simulink model "six_stepItext"  (R2024a)
settings: Solver=ode23t  StartTime=0.0  StopTime=10  MaxStep=1e-6  RelTol=1e-4
undefined symbols (not defined in the file): DiscIntNeverNeededParam
libraries: simulink x24, nesl_utility x13, ee_lib x6, fl_lib x6, eePwmGenerator x1
(part 1 of 2)
settings Model: SimulationMode=accelerator  Creator=25415  LastModifiedBy=25415

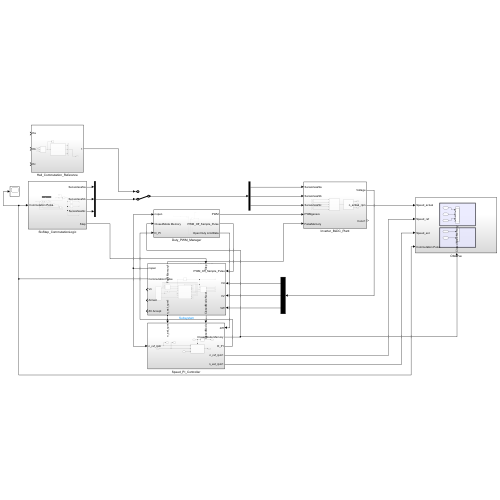
[thumbnail: Simulink's stored preview of the top-level diagram]
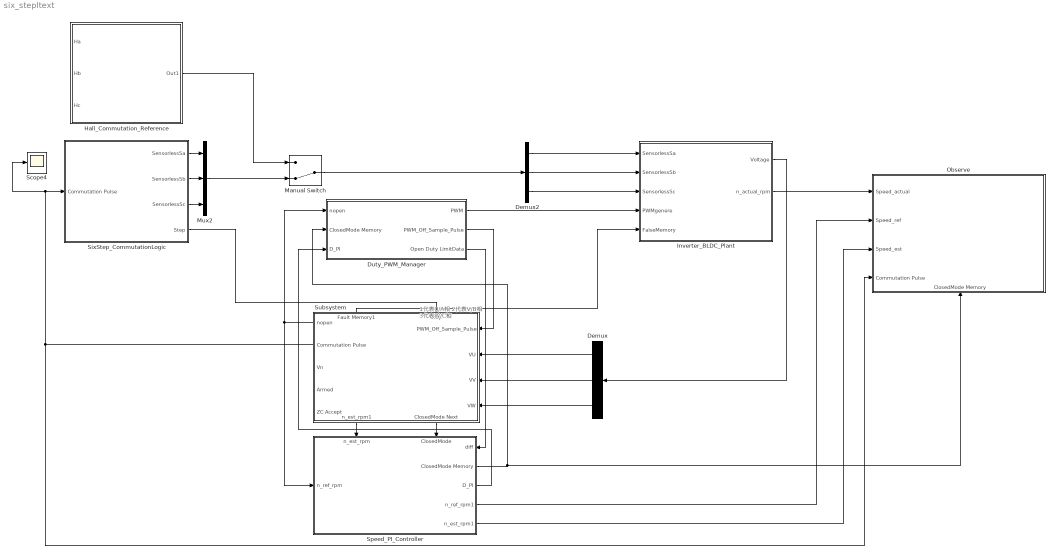
== system six_stepItext ==
  note: 1代表U/A相
      | 2代表V/B相
      | 3代表W/C相
  Demux : Demux  Outputs=3
  Demux2 : Demux  Outputs=3
  Duty_PWM_Manager : Subsystem
  Hall_Commutation_Reference : Subsystem
  Inverter_BLDC_Plant : Subsystem
  Manual Switch : ManualSwitch  CurrentSetting=0
  Mux2 : Mux  Inputs=3
  Observe : Subsystem
      settings: PortSchema="{\"entries\":[{\"content\":{\"sides\":[{\"content\":{\"connectorIds\":[\"In1\",\"In2\",\"In3\",\"In4\"]},\"type\":\"ConnectorPlacement.EquallySpacedRectSide\",\"uuid\":\"9088793b-2014-4196-a719-1ae128c634bd\"},{\"content\":{\"side\":\"RIGHT\"},\"type\":\"ConnectorPlacement.EquallySpacedRectSide\",\"uuid\":\"173c01ed-895e-413e-a79c-9815030dd1a7\"},{\"content\":{\"side\":\"TOP\"},\"type\":\"ConnectorPlacement.EquallySpacedRectSide\",\"uuid\":\"97f01aa3-a0bc-4305-9aad-804b5494463d\"},{\"content\":{\"connectorIds\":[\"In5\"],\"side\":\"BOTTOM\"},\"type\":\"ConnectorPlacement.EquallySpacedRectSide\",\"uuid\":\"39a9b1ee-11d5-4763-bc6a-eddc1daf8ee3\"}]},\"type\":\"ConnectorPlacement.EquallySpacedConnector\",\"uuid\":\"f0f9deaa-30fa-496c-8cff-10ccb2f5b2cf\"}],\"packageUris\":[\"http://schema.mathworks.com/mf0/Connector/R2020b\"],\"version\":\"1.0\"}"
  Scope4 : Scope
  SixStep_CommutationLogic : Subsystem
  Speed_PI_Controller : Subsystem
      settings: PortSchema="{\"entries\":[{\"content\":{\"sides\":[{\"content\":{\"connectorIds\":[\"In1\"]},\"type\":\"ConnectorPlacement.EquallySpacedRectSide\",\"uuid\":\"8a8ee2e6-da43-4c48-942d-e921ad8bcf3e\"},{\"content\":{\"connectorIds\":[\"In4\",\"Out1\",\"Out2\",\"Out3\",\"Out4\"],\"side\":\"RIGHT\"},\"type\":\"ConnectorPlacement.EquallySpacedRectSide\",\"uuid\":\"836c52b4-ac3a-4487-9ffc-d5efd4795786\"},{\"content\":{\"connectorIds\":[\"In2\",\"In3\"],\"side\":\"TOP\"},\"type\":\"ConnectorPlacement.EquallySpacedRectSide\",\"uuid\":\"5ec63cd2-cc9c-4304-9815-6f512e278e15\"},{\"content\":{\"side\":\"BOTTOM\"},\"type\":\"ConnectorPlacement.EquallySpacedRectSide\",\"uuid\":\"5132e6d1-af86-4b59-9d6a-b07b9b3af0b9\"}]},\"type\":\"ConnectorPlacement.EquallySpacedConnector\",\"uuid\":\"ac3d9a82-96c0-4f89-ae52-07d69004cd78\"}],\"packageUris\":[\"http://schema.mathworks.com/mf0/Connector/R2020b\"],\"version\":\"1.0\"}"
  Subsystem : Subsystem
      settings: PortSchema="{\"entries\":[{\"content\":{\"sides\":[{\"content\":{\"connectorIds\":[\"In1\",\"In2\",\"In3\",\"In4\"]},\"type\":\"ConnectorPlacement.EquallySpacedRectSide\",\"uuid\":\"0454e366-7b0d-4657-8f1b-5f34838f4f79\"},{\"content\":{\"connectorIds\":[\"Out1\",\"Out2\",\"Out3\",\"Out4\",\"Out5\"],\"side\":\"RIGHT\"},\"type\":\"ConnectorPlacement.EquallySpacedRectSide\",\"uuid\":\"85c00b62-bded-4496-b2c0-b773fc71ee5c\"},{\"content\":{\"connectorIds\":[\"In5\",\"Out8\"],\"side\":\"TOP\"},\"type\":\"ConnectorPlacement.EquallySpacedRectSide\",\"uuid\":\"3240dca5-fa46-4bda-9873-c5e2b8c1d629\"},{\"content\":{\"connectorIds\":[\"Out6\",\"Out7\"],\"side\":\"BOTTOM\"},\"type\":\"ConnectorPlacement.EquallySpacedRectSide\",\"uuid\":\"47798f7f-7eed-4b14-9289-d21656a674be\"}]},\"type\":\"ConnectorPlacement.EquallySpacedConnector\",\"uuid\":\"b9e37fa7-d7c3-43fc-b27e-fc50c7c41c36\"}],\"packageUris\":[\"http://schema.mathworks.com/mf0/Connector/R2020b\"],\"version\":\"1.0\"}"
  wires:
  SixStep_CommutationLogic/2(SensorlessSb) -> Mux2/2
  SixStep_CommutationLogic/1(SensorlessSa) -> Mux2/1
  SixStep_CommutationLogic/3(SensorlessSc) -> Mux2/3
  Mux2/1 -> Manual Switch/2
  Hall_Commutation_Reference/1(Out1) -> Manual Switch/1
  Manual Switch/1 -> Demux2/1
  Demux2/1 -> Inverter_BLDC_Plant/1(SensorlessSa)
  Demux2/2 -> Inverter_BLDC_Plant/2(SensorlessSb)
  Demux2/3 -> Inverter_BLDC_Plant/3(SensorlessSc)
  Inverter_BLDC_Plant/1(Voltage) -> Demux/1
  Duty_PWM_Manager/1(PWM) -> Inverter_BLDC_Plant/4(PWMgenere)
  Duty_PWM_Manager/3(Open Duty LimitData) -> Speed_PI_Controller/4(diff)
  Speed_PI_Controller/1(ClosedMode Memory) -> Observe/5(ClosedMode Memory), Duty_PWM_Manager/2(ClosedMode Memory)
  Speed_PI_Controller/2(D_PI) -> Duty_PWM_Manager/3(D_PI)
  Subsystem/2(Commutation Pulse) -> Scope4/1, SixStep_CommutationLogic/1(Commutation Pulse), Observe/4(Commutation Pulse)
  Subsystem/1(nopen) -> Duty_PWM_Manager/1(nopen), Speed_PI_Controller/1(n_ref_rpm)
  Duty_PWM_Manager/2(PWM_Off_Sample_Pulse) -> Subsystem/1(PWM_Off_Sample_Pulse)
  SixStep_CommutationLogic/4(Step) -> Subsystem/5(Step)
  Demux/1 -> Subsystem/2(VU)
  Demux/2 -> Subsystem/3(VV)
  Demux/3 -> Subsystem/4(VW)
  Subsystem/8(Fault Memory1) -> Inverter_BLDC_Plant/5(FalseMemory)
  Subsystem/6(ClosedMode Next) -> Speed_PI_Controller/3(ClosedMode)
  Subsystem/7(n_est_rpm1) -> Speed_PI_Controller/2(n_est_rpm)
  Speed_PI_Controller/3(n_ref_rpm1) -> Observe/2(Speed_ref)
  Speed_PI_Controller/4(n_est_rpm1) -> Observe/3(Speed_est)
  Inverter_BLDC_Plant/2(n_actual_rpm) -> Observe/1(Speed_actual)

== system six_stepItext/Duty_PWM_Manager ==
  nopen : Inport
  ClosedMode Memory : Inport  Port=2
  D_PI : Inport  Port=3
  Detect Decrease : simulink/Logic and Bit Operations/Detect Decrease  vinit=0.0  OutDataTypeStr=boolean
  Subsystem : Subsystem
  Subsystem3 : Subsystem
  Unit Delay : UnitDelay  SampleTime=10e-6  HasFrameUpgradeWarning=on
  Zero-Order Hold1 : ZeroOrderHold  SampleTime=10e-6
  PWM : Outport
  PWM_Off_Sample_Pulse : Outport  Port=2
  Open Duty LimitData : Outport  Port=3
  wires:
  D_PI/1 -> Subsystem3/3(D_PI)
  Subsystem3/1(PWM) -> PWM/1, Zero-Order Hold1/1
  ClosedMode Memory/1 -> Subsystem3/2(ClosedMode Memory)
  Subsystem/1(Open Duty LimitData) -> Open Duty LimitData/1, Subsystem3/1(In1)
  Zero-Order Hold1/1 -> Detect Decrease/1  "PWM_10us"
  Detect Decrease/1 -> Unit Delay/1
  nopen/1 -> Subsystem/1(nopen)
  Unit Delay/1 -> PWM_Off_Sample_Pulse/1  "PWM_Off_Sample_Pulse"

== system six_stepItext/Hall_Commutation_Reference ==
  Ha : Inport
  Hb : Inport  Port=2
  Hc : Inport  Port=3
  Hallencoder : Subsystem
  Mux1 : Mux  Inputs=3
  Scope2 : Scope
  Subsystem : Subsystem
  Out1 : Outport
  wires:
  Hb/1 -> Hallencoder/2(Hb)
  Subsystem/2(Sb) -> Mux1/2
  Subsystem/1(Sa) -> Mux1/1
  Mux1/1 -> Out1/1
  Hallencoder/1(Hallcode) -> Scope2/1, Subsystem/1(Hallcode)
  Hc/1 -> Hallencoder/3(Hc)
  Subsystem/3(Sc) -> Mux1/3
  Ha/1 -> Hallencoder/1(Ha)

== system six_stepItext/Inverter_BLDC_Plant ==
  SensorlessSa : Inport
  SensorlessSb : Inport  Port=2
  SensorlessSc : Inport  Port=3
  PWMgenere : Inport  Port=4
  FalseMemory : Inport  Port=5
  DriveSystem : Subsystem
  Subsystem2 : Subsystem
  Conn1 : PMIOPort  Side=Right
  Voltage : Outport
  n_actual_rpm : Outport  Port=2
  wires:
  SensorlessSc/1 -> DriveSystem/3(SensorlessSc)
  Subsystem2/1(Voltage) -> Voltage/1
  FalseMemory/1 -> DriveSystem/5(FalseMemory)
  PWMgenere/1 -> DriveSystem/4(PWMgenere)
  SensorlessSa/1 -> DriveSystem/1(SensorlessSa)
  SensorlessSb/1 -> DriveSystem/2(SensorlessSb)
  Subsystem2/2(n_actual_rpm) -> n_actual_rpm/1
  connections:
  Subsystem2/RConn1 -- Conn1/RConn1
  DriveSystem/RConn1 -- Subsystem2/LConn1

== system six_stepItext/Observe ==
  note: SpeedObserve
  note: StateObserve
  Speed_actual : Inport
  Speed_ref : Inport  Port=2
  Speed_est : Inport  Port=3
  Commutation Pulse : Inport  Port=4
  ClosedMode Memory : Inport  Port=5
  Scope : Scope  NumInputPorts=3
  Scope1 : Scope  NumInputPorts=2
  Scope2 : Scope  NumInputPorts=3
  wires:
  Speed_ref/1 -> Scope/1
  Speed_est/1 -> Scope/2
  Speed_actual/1 -> Scope/3
  Commutation Pulse/1 -> Scope1/1
  ClosedMode Memory/1 -> Scope1/2

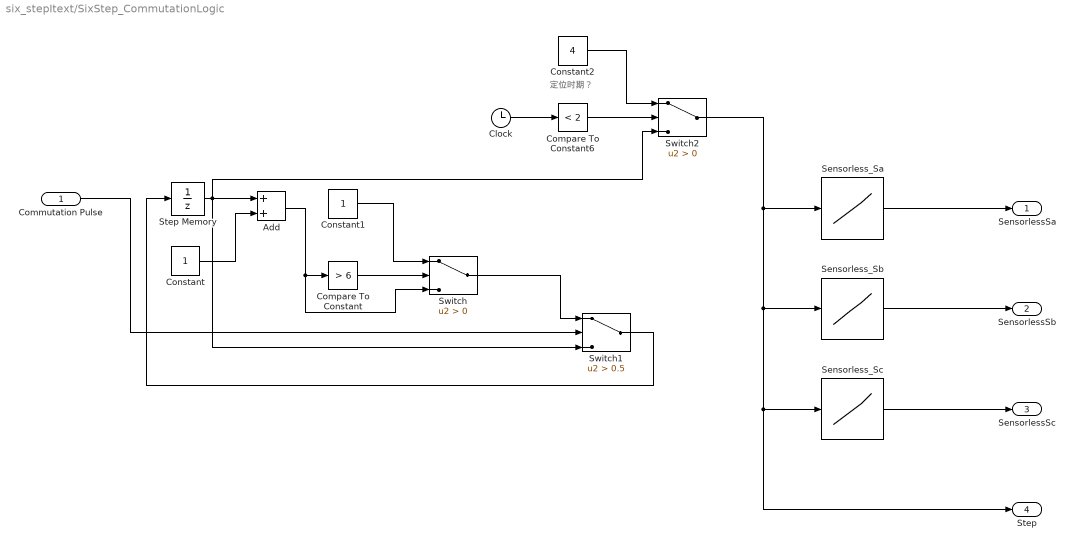
== system six_stepItext/SixStep_CommutationLogic ==
  note: 定位时期？
  Commutation Pulse : Inport
  Add : Sum
  Clock : Clock
  Compare To Constant : simulink/Logic and Bit Operations/Compare To Constant  relop=>  const=6  OutDataTypeStr=boolean
  Compare To Constant6 : simulink/Logic and Bit Operations/Compare To Constant  relop=<  const=2  OutDataTypeStr=boolean
  Constant : Constant
  Constant1 : Constant
  Constant2 : Constant  Value=4
  Sensorless_Sa : Lookup_n-D  NumberOfTableDimensions=1  BreakpointsForDimension1=[0 1 2 3 4 5 6]  Table=[0 -1 -1 0 1 1 0]  InterpMethod=Flat  InternalRulePriority=Speed  OutDataTypeStr=double  RndMeth=Simplest
  Sensorless_Sb : Lookup_n-D  NumberOfTableDimensions=1  BreakpointsForDimension1=[0 1 2 3 4 5 6]  Table=[0 1 0 -1 -1 0 1]  InterpMethod=Flat  InternalRulePriority=Speed  OutDataTypeStr=double  RndMeth=Simplest
  Sensorless_Sc : Lookup_n-D  NumberOfTableDimensions=1  BreakpointsForDimension1=[0 1 2 3 4 5 6]  Table=[0 0 1 1 0 -1 -1]  InterpMethod=Flat  InternalRulePriority=Speed  OutDataTypeStr=double  RndMeth=Simplest
  Step Memory : UnitDelay  InitialCondition=5  SampleTime=10e-6  HasFrameUpgradeWarning=on
  Switch : Switch  Criteria=u2 > Threshold  SaturateOnIntegerOverflow=off  InputSameDT=off
  Switch1 : Switch  Criteria=u2 > Threshold  Threshold=0.5  SaturateOnIntegerOverflow=off  InputSameDT=off
  Switch2 : Switch  Criteria=u2 > Threshold  SaturateOnIntegerOverflow=off  InputSameDT=off
  SensorlessSa : Outport
  SensorlessSb : Outport  Port=2
  SensorlessSc : Outport  Port=3
  Step : Outport  Port=4
  wires:
  Step Memory/1 -> Add/1, Switch2/3, Switch1/3
  Constant/1 -> Add/2
  Add/1 -> Switch/3, Compare To Constant/1
  Compare To Constant/1 -> Switch/2
  Constant1/1 -> Switch/1
  Commutation Pulse/1 -> Switch1/2
  Switch1/1 -> Step Memory/1
  Sensorless_Sa/1 -> SensorlessSa/1
  Sensorless_Sb/1 -> SensorlessSb/1
  Sensorless_Sc/1 -> SensorlessSc/1
  Clock/1 -> Compare To Constant6/1
  Compare To Constant6/1 -> Switch2/2
  Constant2/1 -> Switch2/1
  Switch/1 -> Switch1/1
  Switch2/1 -> Sensorless_Sa/1, Sensorless_Sb/1, Step/1, Sensorless_Sc/1

== system six_stepItext/Speed_PI_Controller ==
  n_ref_rpm : Inport
  n_est_rpm : Inport  Port=2
  ClosedMode : Inport  Port=3
  diff : Inport  Port=4
  ClosedMode Memory1 : UnitDelay  SampleTime=10e-6  HasFrameUpgradeWarning=on
  Enabled Subsystem : Subsystem  TreatAsAtomicUnit=on
  ClosedMode Memory : Outport
  D_PI : Outport  Port=2
  n_ref_rpm1 : Outport  Port=3
  n_est_rpm1 : Outport  Port=4
  wires:
  diff/1 -> Enabled Subsystem/3(diff)
  n_ref_rpm/1 -> n_ref_rpm1/1, Enabled Subsystem/1(n_ref_rpm)
  ClosedMode/1 -> ClosedMode Memory1/1, Enabled Subsystem/Enable
  Enabled Subsystem/1(D_PI) -> D_PI/1
  ClosedMode Memory1/1 -> ClosedMode Memory/1
  n_est_rpm/1 -> n_est_rpm1/1, Enabled Subsystem/2(n_fb_rpm)

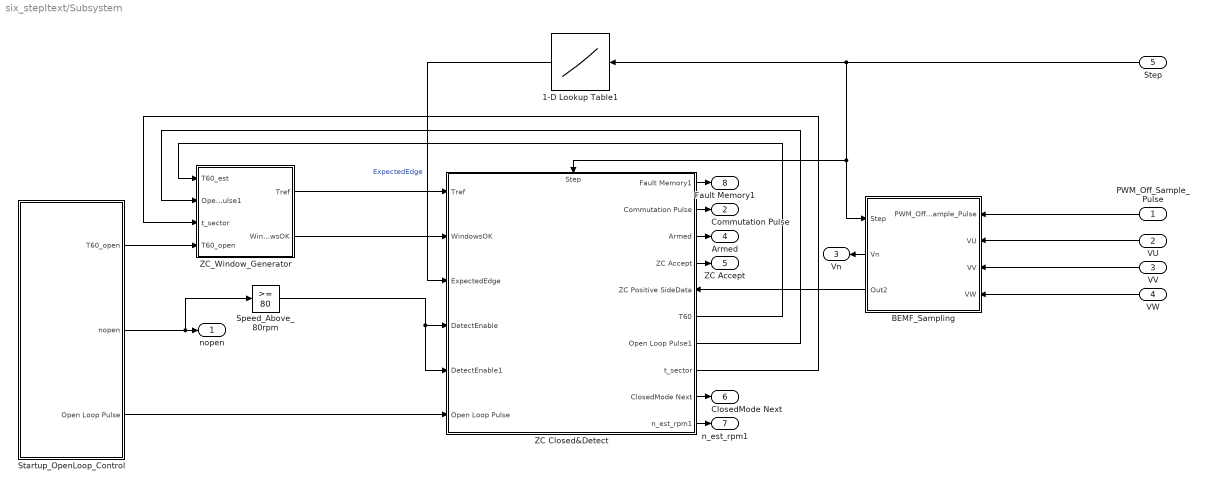
== system six_stepItext/Subsystem ==
  PWM_Off_Sample_Pulse : Inport
  VU : Inport  Port=2
  VV : Inport  Port=3
  VW : Inport  Port=4
  Step : Inport  Port=5
  1-D Lookup Table1 : Lookup_n-D  NumberOfTableDimensions=1  BreakpointsForDimension1=[0 1 2 3 4 5 6]  Table=[0 1 0 1 0 1 0]  InterpMethod=Flat  InternalRulePriority=Speed  RndMeth=Simplest
  BEMF_Sampling : Subsystem
      settings: PortSchema="{\"entries\":[{\"content\":{\"sides\":[{\"content\":{\"connectorIds\":[\"In1\",\"In2\",\"In3\",\"In4\"]},\"type\":\"ConnectorPlacement.EquallySpacedRectSide\",\"uuid\":\"219db874-4903-4521-ac7a-a4e5cace14e3\"},{\"content\":{\"connectorIds\":[\"In5\",\"Out1\",\"Out2\"],\"side\":\"RIGHT\"},\"type\":\"ConnectorPlacement.EquallySpacedRectSide\",\"uuid\":\"060f3999-5577-4659-ac56-31576aafd858\"},{\"content\":{\"side\":\"TOP\"},\"type\":\"ConnectorPlacement.EquallySpacedRectSide\",\"uuid\":\"b4eedb8b-4b2d-4953-a2bb-d0f589dd93bb\"}]},\"type\":\"ConnectorPlacement.EquallySpacedConnector\",\"uuid\":\"c9675ca2-e6a6-43e7-bc9f-5a6e20bc96da\"}],\"packageUris\":[\"http://schema.mathworks.com/mf0/Connector/R2020b\"],\"version\":\"1.0\"}"
  Speed_Above_80rpm : simulink/Logic and Bit Operations/Compare To Constant  relop=>=  const=80  OutDataTypeStr=boolean
  Startup_OpenLoop_Control : Subsystem
  ZC Closed&Detect : Subsystem
      settings: PortSchema="{\"entries\":[{\"content\":{\"sides\":[{\"content\":{\"connectorIds\":[\"In1\",\"In2\",\"In3\",\"In4\",\"In5\",\"In6\"]},\"type\":\"ConnectorPlacement.EquallySpacedRectSide\",\"uuid\":\"236afadc-2b12-4f95-9b78-5ff144fef5c1\"},{\"content\":{\"connectorIds\":[\"Out1\",\"Out2\",\"Out3\",\"Out4\",\"In8\",\"Out5\",\"Out6\",\"Out7\",\"Out8\",\"Out9\"],\"side\":\"RIGHT\"},\"type\":\"ConnectorPlacement.EquallySpacedRectSide\",\"uuid\":\"406734ed-d81f-414f-95f5-b90d5cc47299\"},{\"content\":{\"connectorIds\":[\"In7\"],\"side\":\"TOP\"},\"type\":\"ConnectorPlacement.EquallySpacedRectSide\",\"uuid\":\"56c21215-f7ac-4aca-9a8a-3ea4f76aa518\"}]},\"type\":\"ConnectorPlacement.EquallySpacedConnector\",\"uuid\":\"992103e6-5b89-45d8-b138-c7ecb7c3dad5\"}],\"packageUris\":[\"http://schema.mathworks.com/mf0/Connector/R2020b\"],\"version\":\"1.0\"}"
  ZC_Window_Generator : Subsystem
  nopen : Outport
  Commutation Pulse : Outport  Port=2
  Vn : Outport  Port=3
  Armed : Outport  Port=4
  ZC Accept : Outport  Port=5
  ClosedMode Next : Outport  Port=6
  n_est_rpm1 : Outport  Port=7
  Fault Memory1 : Outport  Port=8
  wires:
  ZC_Window_Generator/2(WindowsOK) -> ZC Closed&Detect/2(WindowsOK)
  Step/1 -> BEMF_Sampling/5(Step), ZC Closed&Detect/7(Step), 1-D Lookup Table1/1
  BEMF_Sampling/1(Vn) -> Vn/1
  ZC Closed&Detect/5(T60) -> ZC_Window_Generator/1(T60_est)
  Startup_OpenLoop_Control/1(T60_open) -> ZC_Window_Generator/4(T60_open)
  BEMF_Sampling/2(Out2) -> ZC Closed&Detect/8(ZC Positive SideData)
  Startup_OpenLoop_Control/3(Open Loop Pulse) -> ZC Closed&Detect/6(Open Loop Pulse)
  ZC Closed&Detect/7(t_sector) -> ZC_Window_Generator/3(t_sector)
  1-D Lookup Table1/1 -> ZC Closed&Detect/3(ExpectedEdge)  "ExpectedEdge"
  ZC Closed&Detect/9(n_est_rpm1) -> n_est_rpm1/1
  ZC Closed&Detect/6(Open Loop Pulse1) -> ZC_Window_Generator/2(Open Loop Pulse1)
  ZC_Window_Generator/1(Tref) -> ZC Closed&Detect/1(Tref)
  VW/1 -> BEMF_Sampling/4(VW)
  VU/1 -> BEMF_Sampling/2(VU)
  PWM_Off_Sample_Pulse/1 -> BEMF_Sampling/1(PWM_Off_Sample_Pulse)
  VV/1 -> BEMF_Sampling/3(VV)
  ZC Closed&Detect/2(Commutation Pulse) -> Commutation Pulse/1
  Startup_OpenLoop_Control/2(nopen) -> Speed_Above_80rpm/1, nopen/1
  ZC Closed&Detect/8(ClosedMode Next) -> ClosedMode Next/1
  ZC Closed&Detect/1(Fault Memory1) -> Fault Memory1/1
  ZC Closed&Detect/3(Armed) -> Armed/1
  ZC Closed&Detect/4(ZC Accept) -> ZC Accept/1
  Speed_Above_80rpm/1 -> ZC Closed&Detect/5(DetectEnable1), ZC Closed&Detect/4(DetectEnable)

== system six_stepItext/Duty_PWM_Manager/Subsystem ==
  nopen : Inport
  Add : Sum
  Divide : Product  Inputs=*/
  Open DC Voltage : Constant  Value=12
  Open Duty Limit : Saturate  UpperLimit=0.45  LowerLimit=0
  Open EMF Voltage : Gain  Gain=0.032
  Open Voltage Boost : Constant  Value=0.4
  Open Duty LimitData : Outport
  wires:
  Divide/1 -> Open Duty Limit/1
  Open DC Voltage/1 -> Divide/2
  Add/1 -> Divide/1
  Open Voltage Boost/1 -> Add/2
  Open EMF Voltage/1 -> Add/1
  Open Duty Limit/1 -> Open Duty LimitData/1
  nopen/1 -> Open EMF Voltage/1

== system six_stepItext/Duty_PWM_Manager/Subsystem3 ==
  In1 : Inport
  ClosedMode Memory : Inport  Port=2
  D_PI : Inport  Port=3
  Clock : Clock
  Compare To Constant7 : simulink/Logic and Bit Operations/Compare To Constant  relop=<  const=2  OutDataTypeStr=boolean
  Constant : Constant  Value=0.05
  PWM Generator : eePwmGenerator/PWM Generator  CarrCount=Up  Tper=50e-6  Tdelay=0  Ts=1e-6
  Subsystem2 : Subsystem
  Switch1 : Switch  Criteria=u2 > Threshold  SaturateOnIntegerOverflow=off  InputSameDT=off
  PWM : Outport
  wires:
  Constant/1 -> Switch1/1
  D_PI/1 -> Subsystem2/1(D_PI)
  Switch1/1 -> Subsystem2/3(Duty)
  Clock/1 -> Compare To Constant7/1
  Compare To Constant7/1 -> Switch1/2
  ClosedMode Memory/1 -> Subsystem2/2(ClosedMode Memory)
  Subsystem2/1(PWM Generator) -> PWM Generator/1
  In1/1 -> Switch1/3
  PWM Generator/1 -> PWM/1

== system six_stepItext/Hall_Commutation_Reference/Hallencoder ==
  Ha : Inport
  Hb : Inport  Port=2
  Hc : Inport  Port=3
  Add : Sum  Inputs=+++
  Gain : Gain  Gain=4
  Gain1 : Gain  Gain=2
  Gain2 : Gain
  Hallcode : Outport
  wires:
  Ha/1 -> Gain/1
  Hc/1 -> Gain2/1
  Hb/1 -> Gain1/1
  Gain/1 -> Add/1
  Gain1/1 -> Add/2
  Gain2/1 -> Add/3
  Add/1 -> Hallcode/1

== system six_stepItext/Hall_Commutation_Reference/Subsystem ==
  Hallcode : Inport
  1-D Lookup Table : Lookup_n-D  NumberOfTableDimensions=1  BreakpointsForDimension1=[0 1 2 3 4 5 6 7]  Table=[0 0 -1 -1 1 1 0 0]  InterpMethod=Flat  InternalRulePriority=Speed  OutDataTypeStr=double  RndMeth=Simplest
  1-D Lookup Table1 : Lookup_n-D  NumberOfTableDimensions=1  BreakpointsForDimension1=[0 1 2 3 4 5 6 7]  Table=[0 -1 1 0 0 -1 1 0]  InterpMethod=Flat  InternalRulePriority=Speed  OutDataTypeStr=double  RndMeth=Simplest
  1-D Lookup Table2 : Lookup_n-D  NumberOfTableDimensions=1  BreakpointsForDimension1=[0 1 2 3 4 5 6 7]  Table=[0 1 0 1 -1 0 -1 0]  InterpMethod=Flat  InternalRulePriority=Speed  OutDataTypeStr=double  RndMeth=Simplest
  Sa : Outport
  Sb : Outport  Port=2
  Sc : Outport  Port=3
  wires:
  Hallcode/1 -> 1-D Lookup Table2/1, 1-D Lookup Table1/1, 1-D Lookup Table/1
  1-D Lookup Table/1 -> Sa/1
  1-D Lookup Table1/1 -> Sb/1
  1-D Lookup Table2/1 -> Sc/1

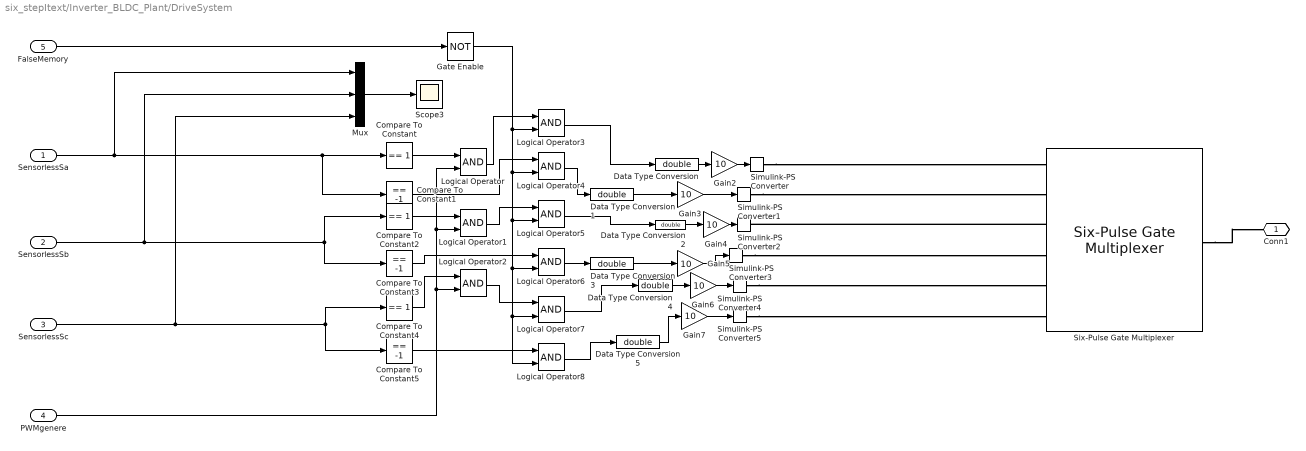
== system six_stepItext/Inverter_BLDC_Plant/DriveSystem ==
  SensorlessSa : Inport
  SensorlessSb : Inport  Port=2
  SensorlessSc : Inport  Port=3
  PWMgenere : Inport  Port=4
  FalseMemory : Inport  Port=5
  Compare To Constant : simulink/Logic and Bit Operations/Compare To Constant  relop===  const=1  OutDataTypeStr=boolean
  Compare To Constant1 : simulink/Logic and Bit Operations/Compare To Constant  relop===  const=-1  OutDataTypeStr=boolean
  Compare To Constant2 : simulink/Logic and Bit Operations/Compare To Constant  relop===  const=1  OutDataTypeStr=boolean
  Compare To Constant3 : simulink/Logic and Bit Operations/Compare To Constant  relop===  const=-1  OutDataTypeStr=boolean
  Compare To Constant4 : simulink/Logic and Bit Operations/Compare To Constant  relop===  const=1  OutDataTypeStr=boolean
  Compare To Constant5 : simulink/Logic and Bit Operations/Compare To Constant  relop===  const=-1  OutDataTypeStr=boolean
  Data Type Conversion{,1..5} (6 alike) : DataTypeConversion  OutDataTypeStr=double  SaturateOnIntegerOverflow=off  RndMeth=Floor
  Gain{2..7} (6 alike) : Gain  Gain=10
  Gate Enable : Logic  Operator=NOT  AllPortsSameDT=off  OutDataTypeStr=boolean
  Logical Operator{,1..8} (9 alike) : Logic  AllPortsSameDT=off  OutDataTypeStr=boolean
  Mux : Mux  Inputs=3
  Scope3 : Scope
  Simulink-PS Converter{,1..5} (6 alike) : nesl_utility/Simulink-PS Converter  PhysicalDomain=network_engine_domain  SubClassName=ps_input  LeftPortType=input  RightPortType=output  PseudoPeriodic=off  Frequencies=[]  NoiseDistribution=none  NoiseParameters=[]  Unit=V  AffineConversion=off  FilteringAndDerivatives=zero  SimscapeFilterOrder=1  InputFilterTimeConstant=0.001  UdotUserProvided=0
  Six-Pulse Gate Multiplexer : ee_lib/Semiconductors & Converters/Converters/Six-Pulse Gate Multiplexer  port_option=ee.enum.controlport.ps
  Conn1 : PMIOPort  Side=Right
  wires:
  Gain3/1 -> Simulink-PS Converter1/1
  SensorlessSb/1 -> Mux/2, Compare To Constant3/1, Compare To Constant2/1
  Data Type Conversion4/1 -> Gain6/1
  PWMgenere/1 -> Logical Operator1/2, Logical Operator/2, Logical Operator2/2
  SensorlessSc/1 -> Mux/3, Compare To Constant5/1, Compare To Constant4/1
  Gain2/1 -> Simulink-PS Converter/1
  Data Type Conversion5/1 -> Gain7/1
  Gain4/1 -> Simulink-PS Converter2/1
  Compare To Constant4/1 -> Logical Operator2/1
  Gain5/1 -> Simulink-PS Converter3/1
  Data Type Conversion3/1 -> Gain5/1
  Gain6/1 -> Simulink-PS Converter4/1
  Compare To Constant2/1 -> Logical Operator1/1
  Data Type Conversion/1 -> Gain2/1
  Mux/1 -> Scope3/1
  Data Type Conversion1/1 -> Gain3/1
  Data Type Conversion2/1 -> Gain4/1
  FalseMemory/1 -> Gate Enable/1
  SensorlessSa/1 -> Mux/1, Compare To Constant1/1, Compare To Constant/1
  Compare To Constant/1 -> Logical Operator/1
  Gain7/1 -> Simulink-PS Converter5/1
  Gate Enable/1 -> Logical Operator3/2, Logical Operator4/2, Logical Operator5/2, Logical Operator6/2, Logical Operator7/2, Logical Operator8/2
  Compare To Constant5/1 -> Logical Operator8/1
  Logical Operator8/1 -> Data Type Conversion5/1
  Logical Operator2/1 -> Logical Operator7/1
  Logical Operator7/1 -> Data Type Conversion4/1
  Logical Operator6/1 -> Data Type Conversion3/1
  Compare To Constant3/1 -> Logical Operator6/1
  Logical Operator1/1 -> Logical Operator5/1
  Compare To Constant1/1 -> Logical Operator4/1
  Logical Operator/1 -> Logical Operator3/1
  Logical Operator3/1 -> Data Type Conversion/1
  Logical Operator4/1 -> Data Type Conversion1/1
  Logical Operator5/1 -> Data Type Conversion2/1
  connections:
  Simulink-PS Converter1/RConn1 -- Six-Pulse Gate Multiplexer/LConn2
  Six-Pulse Gate Multiplexer/LConn3 -- Simulink-PS Converter2/RConn1
  Simulink-PS Converter/RConn1 -- Six-Pulse Gate Multiplexer/LConn1
  Simulink-PS Converter3/RConn1 -- Six-Pulse Gate Multiplexer/LConn4
  Simulink-PS Converter4/RConn1 -- Six-Pulse Gate Multiplexer/LConn5
  Simulink-PS Converter5/RConn1 -- Six-Pulse Gate Multiplexer/LConn6
  Six-Pulse Gate Multiplexer/RConn1 -- Conn1/RConn1

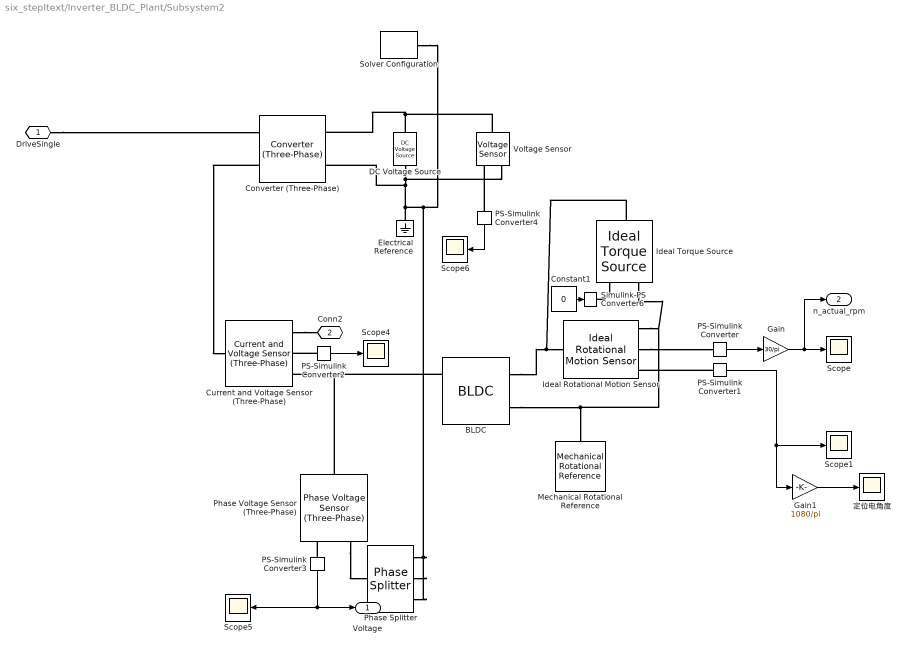
== system six_stepItext/Inverter_BLDC_Plant/Subsystem2 ==
  BLDC : ee_lib/Electromechanical/Permanent Magnet/BLDC  port_option=ee.enum.threePhasePort.composite  rotor_param=ee.enum.pmsm.backemf.trapezoidflux  pm_flux_linkage=0.03 Wb  theta_constant=pi / 12 rad  emf_max=9.6 V  w_meas=600 rpm  DphiDtheta_tab=[0, -.1528, -.1528, .1528, .1528, 0] Wb/rad  back_emf_tab=[0, -9.6, -9.6, 9.6, 9.6, 0] V  rotor_angle_tab=[0, 7.5, 22.5, 37.5, 52.5, 60] deg  nPolePairs=6  axes_param=ee.enum.rotorangle.daxis  winding_type=ee.enum.electromech.statorconfiguration.wye  stator_param=ee.enum.statorparam.LdLqL0  machine_param=ee.enum.dqparameterization.constant  Ld=0.00022 H  Lq=0.00022 H  idVec=[-200, 0, 200] A  iqVec=[-200, 0, 200] A  LdMatrix=0.00022 * ones(3, 3) H  LqMatrix=0.00022 * ones(3, 3) H  L0=0.00016 H  Ls=0.0002 H  Lm=0 H  Ms=0.00002 H  Rs=0.013 Ohm  zero_sequence=ee.enum.park.zerosequence.include  loss_param=ee.enum.ironloss.none  losses_oc=[0, 0, 0] W  losses_sc=[0, 0, 0] W  f_losses=60 Hz  Isc_losses=95 A  J=0.01 kg*m^2  lam=0.05 N*m*s/rad  i_d_specify=off  i_d_priority=None  i_d=0 A  i_d_nominal_specify=off  i_d_nominal_value=1  i_d_nominal_unit=A  i_q_specify=off  i_q_priority=None  i_q=0 A  i_q_nominal_specify=off  i_q_nominal_value=1  i_q_nominal_unit=A  torque_specify=off  torque_priority=None  torque=0 N*m  torque_nominal_specify=off  torque_nominal_value=1  torque_nominal_unit=N*m  angular_velocity_specify=off  angular_velocity_priority=High  angular_velocity=0 rpm  angular_velocity_nominal_specify=off  angular_velocity_nominal_value=1  angular_velocity_nominal_unit=rpm  angular_position_specify=off  angular_position_priority=High  angular_position=0 deg  angular_position_nominal_specify=off  angular_position_nominal_value=1  angular_position_nominal_unit=deg  alpha=3.93e-3 1/K  alpha_flux=-0.001 1/K  Tmeas=298.15 K  stator_thermal_mass=100 J/K  rotor_thermal_mass=200 J/K  Rm_percent_rotor=90  Rd_percent_rotor=30  temperatureA_specify=off  temperatureA_priority=High  temperatureA=25 degC  temperatureA_nominal_specify=off  temperatureA_nominal_value=1  temperatureA_nominal_unit=degC  temperatureB_specify=off  temperatureB_priority=High  temperatureB=25 degC  temperatureB_nominal_specify=off  temperatureB_nominal_value=1  temperatureB_nominal_unit=degC  temperatureC_specify=off  temperatureC_priority=High  temperatureC=25 degC  temperatureC_nominal_specify=off  temperatureC_nominal_value=1  temperatureC_nominal_unit=degC  temperatureR_specify=off  temperatureR_priority=High  temperatureR=25 degC  temperatureR_nominal_specify=off  temperatureR_nominal_value=1  temperatureR_nominal_unit=degC
      settings: InternalSimscapePortConfiguration="{\"Bottom\":[],\"Left\":[{\"id\":\"N\",\"label\":\"~\",\"type\":\"foundation.electrical.three_phase\"},{\"id\":\"n\",\"label\":\"n\",\"type\":\"foundation.electrical.electrical\"}],\"Right\":[{\"id\":\"R\",\"label\":\"R\",\"type\":\"foundation.mechanical.rotational.rotational\"},{\"id\":\"C\",\"label\":\"C\",\"type\":\"foundation.mechanical.rotational.rotational\"}],\"Top\":[]}"
  Constant1 : Constant  Value=0
  Converter (Three-Phase) : ee_lib/Semiconductors & Converters/Converters/Converter (Three-Phase)  port_option=ee.enum.threePhasePort.composite  fidelity_option=ee.enum.converters.fidelity.detailed  device_type=ee.enum.converters.switchingdevice.ideal  K=0  Vf=0.8 V  Ron=0.001 Ohm  Rds=0.001 Ohm  Goff=1e-6 1/Ohm  Vgt=1 V  Vgt_off=-1 V  Ih=1 A  Vth=6 V  diode_param=ee.enum.converters.protectiondiode.nodynamics  diode_Vf=0.8 V  diode_Ron=0.001 Ohm  diode_Goff=1e-5 1/Ohm  diode_C=50 nF  diode_iRM=-235 A  diode_iF=300 A  diode_idot=-50 A/us  diode_trr_param=ee.enum.converters.diodetrr.trr_factor  diode_trr_factor=3  diode_trr=15 us  diode_Qrr=1500 s*uA  snubber_type=ee.enum.converters.snubber.exclude  Cs=1e-7 F  Rs=0.1 Ohm
  Current and Voltage Sensor (Three-Phase) : ee_lib/Sensors & Transducers/Current and Voltage Sensor (Three-Phase)  vMeasurementType=ee.enum.vmeasurement.ll  outputUnit=ee.enum.unit.si  SRated=100e6 A*V  VRated=24e3 V  I_specify=off  I_priority=None  I=[0, 0, 0] A  I_nominal_specify=off  I_nominal_value=1  I_nominal_unit=A  V_specify=off  V_priority=None  V=[0, 0, 0] V  V_nominal_specify=off  V_nominal_value=1  V_nominal_unit=V
      settings: InternalSimscapePortConfiguration="{\"Bottom\":[],\"Left\":[{\"id\":\"N1\",\"label\":\"~1\",\"type\":\"foundation.electrical.three_phase\"}],\"Right\":[{\"id\":\"V_output\",\"label\":\"V\",\"type\":\"output\"},{\"id\":\"I_output\",\"label\":\"I\",\"type\":\"output\"},{\"id\":\"N2\",\"label\":\"~2\",\"type\":\"foundation.electrical.three_phase\"}],\"Top\":[]}"
  DC Voltage Source : fl_lib/Electrical/Electrical Sources/DC Voltage Source  v0=12 V
  Electrical Reference : fl_lib/Electrical/Electrical Elements/Electrical Reference
  Gain : Gain  Gain=30/pi
  Gain1 : Gain  Gain=1080/pi
  Ideal Rotational Motion Sensor : fl_lib/Mechanical/Mechanical Sensors/Ideal Rotational Motion Sensor  reference=foundation.enum.MeasurementReference.difference  acceleration_port=false  velocity_port=true  position_port=true  wrap_angle=false  offset=0 rad
  Ideal Torque Source : fl_lib/Mechanical/Mechanical Sources/Ideal Torque Source
  Mechanical Rotational Reference : fl_lib/Mechanical/Rotational Elements/Mechanical Rotational Reference
  PS-Simulink Converter : nesl_utility/PS-Simulink Converter  PhysicalDomain=network_engine_domain  SubClassName=ps_output  LeftPortType=input  RightPortType=output  PseudoPeriodic=off  Frequencies=[]  VectorFormat=inherit  Unit=rad/s  AffineConversion=off
  PS-Simulink Converter1 : nesl_utility/PS-Simulink Converter  PhysicalDomain=network_engine_domain  SubClassName=ps_output  LeftPortType=input  RightPortType=output  PseudoPeriodic=off  Frequencies=[]  VectorFormat=inherit  Unit=rad  AffineConversion=off
  PS-Simulink Converter2 : nesl_utility/PS-Simulink Converter  PhysicalDomain=network_engine_domain  SubClassName=ps_output  LeftPortType=input  RightPortType=output  PseudoPeriodic=off  Frequencies=[]  VectorFormat=inherit  Unit=A  AffineConversion=off
  PS-Simulink Converter3 : nesl_utility/PS-Simulink Converter  PhysicalDomain=network_engine_domain  SubClassName=ps_output  LeftPortType=input  RightPortType=output  PseudoPeriodic=off  Frequencies=[]  VectorFormat=inherit  Unit=V  AffineConversion=off
  PS-Simulink Converter4 : nesl_utility/PS-Simulink Converter  PhysicalDomain=network_engine_domain  SubClassName=ps_output  LeftPortType=input  RightPortType=output  PseudoPeriodic=off  Frequencies=[]  VectorFormat=inherit  Unit=V  AffineConversion=off
  Phase Splitter : ee_lib/Connectors & References/Phase Splitter
  Phase Voltage Sensor (Three-Phase) : ee_lib/Sensors & Transducers/Phase Voltage Sensor (Three-Phase)
  Scope{,1,4..6} (5 alike) : Scope
  Simulink-PS Converter6 : nesl_utility/Simulink-PS Converter  PhysicalDomain=network_engine_domain  SubClassName=ps_input  LeftPortType=input  RightPortType=output  PseudoPeriodic=off  Frequencies=[]  NoiseDistribution=none  NoiseParameters=[]  Unit=N*m  AffineConversion=off  FilteringAndDerivatives=zero  SimscapeFilterOrder=1  InputFilterTimeConstant=0.001  UdotUserProvided=0
  Solver Configuration : nesl_utility/Solver Configuration  PhysicalDomain=network_engine_domain  SubClassName=solver  LeftPortType=input  RightPortType=generic  Tones=[]  Harmonics=[]  SimulateNoise=off  Profile=off  UseLocalSampling=off  EnableSwitchedLinearOptims=on  FrequencyDomain=off  UseCCode=off  RelTol=0.001  AbsTol=0.001  MinStep=1e-09  ToWorkspace=off  RevertToSquareIcSolve=off  NumHomotopyIterations=100  PhasorMode=off  PhasorModeNumHarmonics=1  ConsistencySolver=NEWTON_XTOL_AFTER_FTOL  IndexReductionMethod=DerivativeReplacement  DoDC=off  ResidualTolerance=1e-09  ConsistencyTolSource=GLOBAL  ConsistencyAbsTol=0.001  ConsistencyRelTol=0.001  ConsistencyTolFactor=0.001  UseLocalSolver=off  LocalSolverChoice=NE_BACKWARD_EULER_ADVANCER  ResolveIndetEquations=on  FunctionEvalNumThread=1  LocalSolverSampleTime=0.001  DoFixedCost=off  MaxNonlinIter=3  MaxModeIter=2  ComputeImpulses=off  ImpulseIterations=2  LinearAlgebra=auto  LinearAlgebraNumThread=0  EquationFormulation=NE_TIME_EF  DelaysMemoryBudget=1024  AutomaticFiltering=on  FilteringTimeConstant=0.001  PartitionStorageMethod=AS_NEEDED  PartitionMemoryBudget=1024  PartitionMethod=ROBUST  MultibodyUseLocalSolver=off  MultibodyLocalSolverChoice=ODE1  MultibodyLocalSolverSampleTime=0.001
  Voltage Sensor : fl_lib/Electrical/Electrical Sensors/Voltage Sensor
  定位电角度 : Scope
  DriveSingle : PMIOPort  Side=Left
  Conn2 : PMIOPort  Port=2  Side=Right
  Voltage : Outport
  n_actual_rpm : Outport  Port=2
  wires:
  PS-Simulink Converter4/1 -> Scope6/1
  PS-Simulink Converter/1 -> Gain/1
  Constant1/1 -> Simulink-PS Converter6/1
  Gain/1 -> n_actual_rpm/1, Scope/1
  PS-Simulink Converter1/1 -> Gain1/1, Scope1/1
  PS-Simulink Converter2/1 -> Scope4/1
  PS-Simulink Converter3/1 -> Voltage/1, Scope5/1
  Gain1/1 -> 定位电角度/1
  connections:
  PS-Simulink Converter3/LConn1 -- Phase Voltage Sensor (Three-Phase)/RConn1
  DC Voltage Source/RConn1 -- Voltage Sensor/RConn2 -- Solver Configuration/RConn1 -- Phase Splitter/RConn3 -- Phase Splitter/RConn2 -- Phase Splitter/RConn1 -- Electrical Reference/LConn1 -- Converter (Three-Phase)/RConn2
  Current and Voltage Sensor (Three-Phase)/RConn1 -- Conn2/RConn1
  BLDC/RConn2 -- Ideal Torque Source/RConn2 -- Ideal Rotational Motion Sensor/RConn1 -- Mechanical Rotational Reference/LConn1
  PS-Simulink Converter1/LConn1 -- Ideal Rotational Motion Sensor/RConn3
  Converter (Three-Phase)/LConn2 -- Current and Voltage Sensor (Three-Phase)/LConn1
  BLDC/LConn1 -- Phase Voltage Sensor (Three-Phase)/LConn1 -- Current and Voltage Sensor (Three-Phase)/RConn3
  DC Voltage Source/LConn1 -- Voltage Sensor/LConn1 -- Converter (Three-Phase)/RConn1
  Phase Voltage Sensor (Three-Phase)/RConn2 -- Phase Splitter/LConn1
  BLDC/RConn1 -- Ideal Torque Source/LConn1 -- Ideal Rotational Motion Sensor/LConn1
  Ideal Rotational Motion Sensor/RConn2 -- PS-Simulink Converter/LConn1
  Ideal Torque Source/RConn1 -- Simulink-PS Converter6/RConn1
  PS-Simulink Converter4/LConn1 -- Voltage Sensor/RConn1
  PS-Simulink Converter2/LConn1 -- Current and Voltage Sensor (Three-Phase)/RConn2
  DriveSingle/RConn1 -- Converter (Three-Phase)/LConn1

== system six_stepItext/Speed_PI_Controller/Enabled Subsystem ==
  n_ref_rpm : Inport
  n_fb_rpm : Inport  Port=2
  diff : Inport  Port=3
  Enable : EnablePort  StatesWhenEnabling=reset
  Add : Sum  Inputs=+-
  Add1 : Sum  Inputs=+++
  Add2 : Sum
  Discrete-Time Integrator1 : DiscreteIntegrator  SampleTime=1e-3  LimitOutput=on  UpperSaturationLimit=0.3  LowerSaturationLimit=-0.3  ICPrevOutput=DiscIntNeverNeededParam  ICPrevScaledInput=DiscIntNeverNeededParam
  KI : Gain  Gain=0.005
  KP : Gain  Gain=0.001
  Kaw : Gain  Gain=5
  Saturation : Saturate  UpperLimit=0.45  LowerLimit=0
  Saturation Error : Sum  Inputs=+-
  D_PI : Outport  OutputWhenDisabled=reset  InitialOutput=0
  wires:
  n_ref_rpm/1 -> Add/1
  n_fb_rpm/1 -> Add/2
  Add/1 -> KP/1, KI/1  "speed_error"
  KI/1 -> Add2/2
  KP/1 -> Add1/1
  Discrete-Time Integrator1/1 -> Add1/2
  diff/1 -> Add1/3
  Add1/1 -> Saturation Error/2, Saturation/1
  Saturation/1 -> Saturation Error/1, D_PI/1
  Saturation Error/1 -> Kaw/1  "speed_error"
  Kaw/1 -> Add2/1
  Add2/1 -> Discrete-Time Integrator1/1  "speed_error"

== system six_stepItext/Subsystem/BEMF_Sampling ==
  note: 在PWM低电平稳定时期采样（实际可以使用PWM中心对齐采样方式）
  PWM_Off_Sample_Pulse : Inport
  VU : Inport  Port=2
  VV : Inport  Port=3
  VW : Inport  Port=4
  Step : Inport  Port=5
  " Floating Phase ID " : Lookup_n-D  NumberOfTableDimensions=1  BreakpointsForDimension1=[0 1 2 3 4 5 6]  Table=[1 3 2 1 3 2 1]  InterpMethod=Flat  InternalRulePriority=Speed  RndMeth=Simplest
  Compute EFloatVolte : Subsystem
  Demux1 : Demux  Outputs=3
  Discrete Filter2 : DiscreteFilter  Numerator=[0.13576]  Denominator=[1 -0.86424]
  Multiport Switch : MultiPortSwitch  SaturateOnIntegerOverflow=off  InputSameDT=off
  Triggered Subsystem : Subsystem  TreatAsAtomicUnit=on
  Zero-Order Hold : ZeroOrderHold  SampleTime=50e-6
  Vn : Outport
  Out2 : Outport  Port=2
  wires:
  Demux1/2 -> Multiport Switch/3
  Demux1/3 -> Multiport Switch/4
  Demux1/1 -> Multiport Switch/2
  Triggered Subsystem/1(Out1) -> Zero-Order Hold/1  "T60raw"
  Discrete Filter2/1 -> Demux1/1
  Multiport Switch/1 -> Out2/1
  " Floating Phase ID "/1 -> Multiport Switch/1
  Zero-Order Hold/1 -> Discrete Filter2/1
  Compute EFloatVolte/2(Eabc) -> Triggered Subsystem/1(Eabc)
  Step/1 -> " Floating Phase ID "/1
  PWM_Off_Sample_Pulse/1 -> Triggered Subsystem/Trigger
  VU/1 -> Compute EFloatVolte/1(VU)
  VV/1 -> Compute EFloatVolte/2(VV)
  VW/1 -> Compute EFloatVolte/3(VW)
  Compute EFloatVolte/1(Vn) -> Vn/1

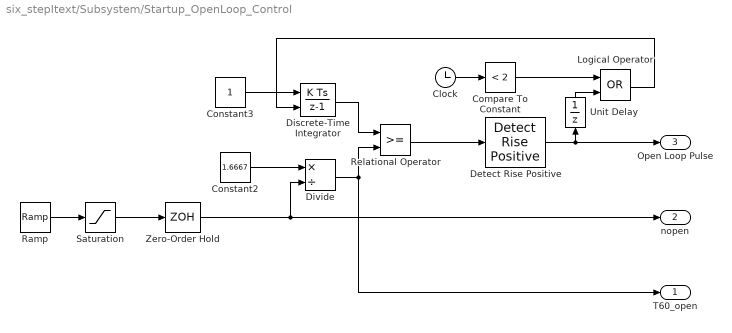
== system six_stepItext/Subsystem/Startup_OpenLoop_Control ==
  Clock : Clock
  Compare To Constant : simulink/Logic and Bit Operations/Compare To Constant  relop=<  const=2  OutDataTypeStr=boolean
  Constant2 : Constant  Value=1.6667
  Constant3 : Constant
  Detect Rise Positive : simulink/Logic and Bit Operations/Detect Rise Positive  vinit=0  OutDataTypeStr=boolean
  Discrete-Time Integrator : DiscreteIntegrator  ExternalReset=level  SampleTime=10e-6  ICPrevOutput=DiscIntNeverNeededParam  ICPrevScaledInput=DiscIntNeverNeededParam
  Divide : Product  Inputs=*/
  Logical Operator : Logic  Operator=OR  AllPortsSameDT=off  OutDataTypeStr=boolean
  Ramp : simulink/Sources/Ramp  slope=20  start=2  InitialOutput=10
  Relational Operator : RelationalOperator  OutDataTypeStr=boolean  RndMeth=Simplest  InputSameDT=off
  Saturation : Saturate  UpperLimit=100  LowerLimit=10
  Unit Delay : UnitDelay  SampleTime=10e-6  HasFrameUpgradeWarning=on
  Zero-Order Hold : ZeroOrderHold  SampleTime=10e-6
  T60_open : Outport
  nopen : Outport  Port=2
  Open Loop Pulse : Outport  Port=3
  wires:
  Constant3/1 -> Discrete-Time Integrator/1
  Saturation/1 -> Zero-Order Hold/1
  Ramp/1 -> Saturation/1
  Constant2/1 -> Divide/1
  Discrete-Time Integrator/1 -> Relational Operator/1
  Divide/1 -> T60_open/1, Relational Operator/2
  Relational Operator/1 -> Detect Rise Positive/1
  Detect Rise Positive/1 -> Unit Delay/1, Open Loop Pulse/1
  Clock/1 -> Compare To Constant/1
  Compare To Constant/1 -> Logical Operator/1
  Logical Operator/1 -> Discrete-Time Integrator/2
  Unit Delay/1 -> Logical Operator/2
  Zero-Order Hold/1 -> nopen/1, Divide/2

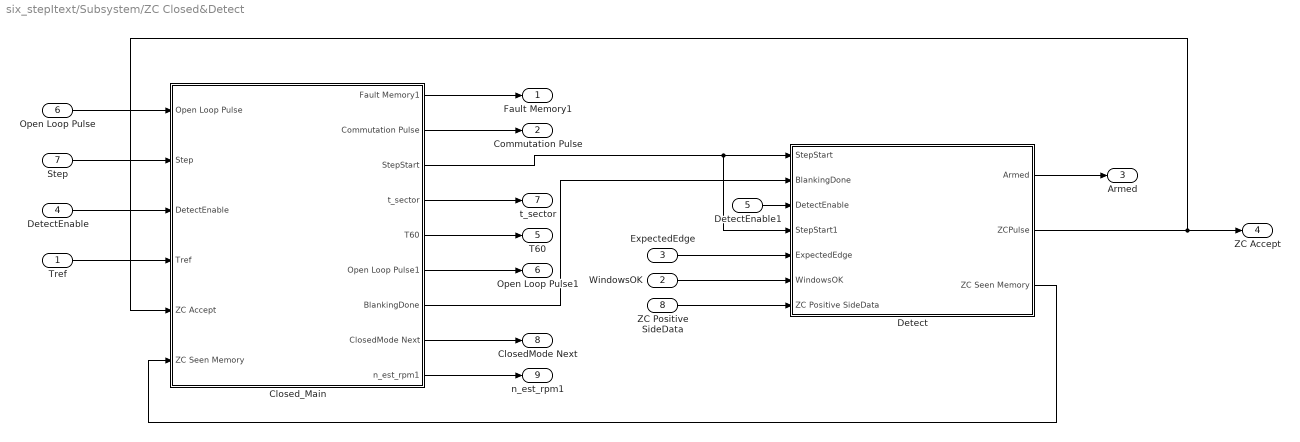
== system six_stepItext/Subsystem/ZC Closed&Detect ==
  Tref : Inport
  WindowsOK : Inport  Port=2
  ExpectedEdge : Inport  Port=3
  DetectEnable : Inport  Port=4
  DetectEnable1 : Inport  Port=5
  Open Loop Pulse : Inport  Port=6
  Step : Inport  Port=7
  ZC Positive SideData : Inport  Port=8
  Closed_Main : Subsystem
  Detect : Subsystem
  Fault Memory1 : Outport
  Commutation Pulse : Outport  Port=2
  Armed : Outport  Port=3
  ZC Accept : Outport  Port=4
  T60 : Outport  Port=5
  Open Loop Pulse1 : Outport  Port=6
  t_sector : Outport  Port=7
  ClosedMode Next : Outport  Port=8
  n_est_rpm1 : Outport  Port=9
  wires:
  Detect/2(ZCPulse) -> Closed_Main/5(ZC Accept), ZC Accept/1
  Closed_Main/1(Fault Memory1) -> Fault Memory1/1
  WindowsOK/1 -> Detect/6(WindowsOK)
  Closed_Main/2(Commutation Pulse) -> Commutation Pulse/1
  ExpectedEdge/1 -> Detect/5(ExpectedEdge)
  Detect/3(ZC Seen Memory) -> Closed_Main/6(ZC Seen Memory)
  Detect/1(Armed) -> Armed/1
  Tref/1 -> Closed_Main/4(Tref)
  Closed_Main/7(BlankingDone) -> Detect/2(BlankingDone)
  Closed_Main/4(t_sector) -> t_sector/1
  ZC Positive SideData/1 -> Detect/7(ZC Positive SideData)
  Closed_Main/5(T60) -> T60/1
  Open Loop Pulse/1 -> Closed_Main/1(Open Loop Pulse)
  Step/1 -> Closed_Main/2(Step)
  Closed_Main/9(n_est_rpm1) -> n_est_rpm1/1
  Closed_Main/8(ClosedMode Next) -> ClosedMode Next/1
  Closed_Main/6(Open Loop Pulse1) -> Open Loop Pulse1/1
  Closed_Main/3(StepStart) -> Detect/4(StepStart1), Detect/1(StepStart)
  DetectEnable/1 -> Closed_Main/3(DetectEnable)
  DetectEnable1/1 -> Detect/3(DetectEnable)

== system six_stepItext/Subsystem/ZC_Window_Generator ==
  T60_est : Inport
  Open Loop Pulse1 : Inport  Port=2
  t_sector : Inport  Port=3
  T60_open : Inport  Port=4
  Gain10 : Gain  Gain=0.75
  Gain9 : Gain  Gain=0.25
  Logical Operator3 : Logic  AllPortsSameDT=off  OutDataTypeStr=boolean
  Relational Operator1 : RelationalOperator  Operator=<=  OutDataTypeStr=boolean  RndMeth=Simplest  InputSameDT=off
  Relational Operator2 : RelationalOperator  OutDataTypeStr=boolean  RndMeth=Simplest  InputSameDT=off
  Switch2 : Switch  Criteria=u2 > Threshold  SaturateOnIntegerOverflow=off  InputSameDT=off
  Tref : Outport
  WindowsOK : Outport  Port=2
  wires:
  Switch2/1 -> Tref/1, Gain9/1, Gain10/1
  Logical Operator3/1 -> WindowsOK/1  "WindowsOK"
  Relational Operator2/1 -> Logical Operator3/1
  Gain10/1 -> Relational Operator1/2
  Relational Operator1/1 -> Logical Operator3/2
  t_sector/1 -> Relational Operator2/1, Relational Operator1/1
  Gain9/1 -> Relational Operator2/2
  Open Loop Pulse1/1 -> Switch2/2
  T60_open/1 -> Switch2/3
  T60_est/1 -> Switch2/1

== system six_stepItext/Duty_PWM_Manager/Subsystem3/Subsystem2 ==
  D_PI : Inport
  ClosedMode Memory : Inport  Port=2
  Duty : Inport  Port=3
  Switch : Switch  Criteria=u2 > Threshold  Threshold=0.5  SaturateOnIntegerOverflow=off  InputSameDT=off
  PWM Generator : Outport
  wires:
  D_PI/1 -> Switch/1
  ClosedMode Memory/1 -> Switch/2
  Duty/1 -> Switch/3
  Switch/1 -> PWM Generator/1

== system six_stepItext/Subsystem/BEMF_Sampling/Compute EFloatVolte ==
  VU : Inport
  VV : Inport  Port=2
  VW : Inport  Port=3
  Constant : Constant  Value=3
  Divide : Product  Inputs=*/
  Mux : Mux  Inputs=3
  Sum : Sum  Inputs=+++
  Sum1 : Sum  Inputs=+-
  Sum2 : Sum  Inputs=+-
  Sum3 : Sum  Inputs=+-
  Vn : Outport
  Eabc : Outport  Port=2
  wires:
  VU/1 -> Sum1/1, Sum/1
  VV/1 -> Sum2/1, Sum/2
  VW/1 -> Sum3/1, Sum/3
  Sum/1 -> Divide/1
  Constant/1 -> Divide/2
  Divide/1 -> Sum1/2, Sum3/2, Sum2/2, Vn/1
  Sum1/1 -> Mux/1
  Sum2/1 -> Mux/2
  Sum3/1 -> Mux/3
  Mux/1 -> Eabc/1

== system six_stepItext/Subsystem/BEMF_Sampling/Triggered Subsystem ==
  Eabc : Inport
  Trigger : TriggerPort  VariantControl=(inherit)
  Out1 : Outport
  wires:
  Eabc/1 -> Out1/1

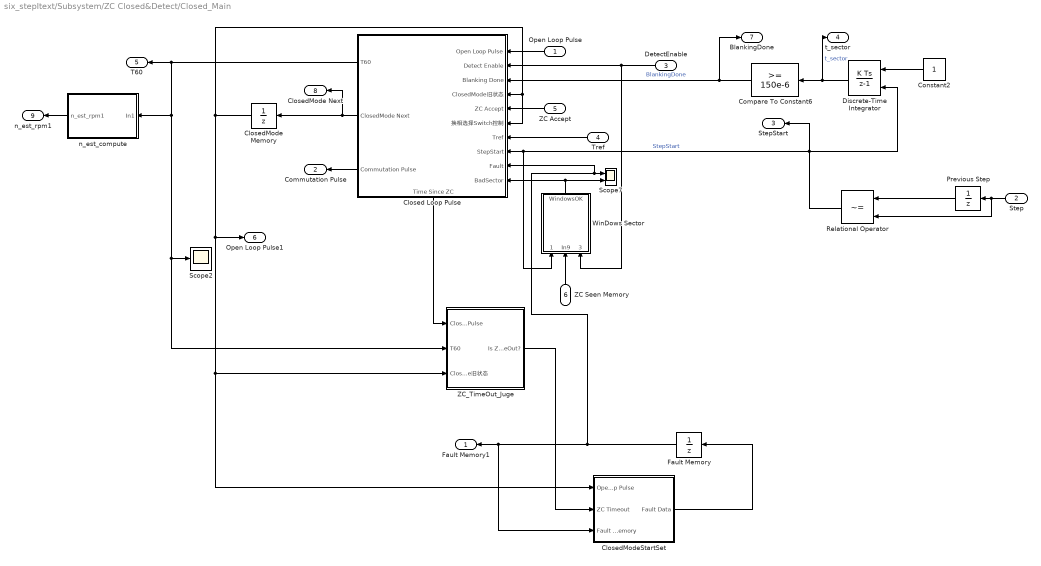
== system six_stepItext/Subsystem/ZC Closed&Detect/Closed_Main ==
  Open Loop Pulse : Inport
  Step : Inport  Port=2
  DetectEnable : Inport  Port=3
  Tref : Inport  Port=4
  ZC Accept : Inport  Port=5
  ZC Seen Memory : Inport  Port=6
  Closed Loop Pulse : Subsystem
      settings: PortSchema="{\"entries\":[{\"content\":{\"sides\":[{\"content\":{\"connectorIds\":[\"In1\",\"In2\",\"In3\",\"In4\",\"In5\",\"In6\",\"In7\",\"In8\",\"In9\",\"In10\"]},\"type\":\"ConnectorPlacement.EquallySpacedRectSide\",\"uuid\":\"4453a6fd-f6d4-44bb-8346-0c1ba2a6940e\"},{\"content\":{\"connectorIds\":[\"Out1\",\"Out2\",\"Out3\"],\"side\":\"RIGHT\"},\"type\":\"ConnectorPlacement.EquallySpacedRectSide\",\"uuid\":\"04620a0b-38ef-4c5f-898f-5f5a569020ce\"},{\"content\":{\"side\":\"TOP\"},\"type\":\"ConnectorPlacement.EquallySpacedRectSide\",\"uuid\":\"73ff148f-ed2c-4028-b0f1-f436aa360de7\"},{\"content\":{\"connectorIds\":[\"Out4\"],\"side\":\"BOTTOM\"},\"type\":\"ConnectorPlacement.EquallySpacedRectSide\",\"uuid\":\"e05072bf-4967-4727-b2ec-05d9e20b254c\"}]},\"type\":\"ConnectorPlacement.EquallySpacedConnector\",\"uuid\":\"96d1c013-4849-40c1-bcef-55b81c521e2c\"}],\"packageUris\":[\"http://schema.mathworks.com/mf0/Connector/R2020b\"],\"version\":\"1.0\"}"
  ClosedMode Memory : UnitDelay  SampleTime=10e-6  HasFrameUpgradeWarning=on
  ClosedModeStartSet : Subsystem
  Compare To Constant6 : simulink/Logic and Bit Operations/Compare To Constant  relop=>=  const=150e-6  OutDataTypeStr=boolean
  Constant2 : Constant
  Discrete-Time Integrator : DiscreteIntegrator  ExternalReset=rising  SampleTime=10e-6  ICPrevOutput=DiscIntNeverNeededParam  ICPrevScaledInput=DiscIntNeverNeededParam
  Fault Memory : UnitDelay  InitialCondition=false  SampleTime=10e-6  HasFrameUpgradeWarning=on
  Previous Step : UnitDelay  InitialCondition=4  SampleTime=10e-6  HasFrameUpgradeWarning=on
  Relational Operator : RelationalOperator  Operator=~=  OutDataTypeStr=boolean  RndMeth=Simplest  InputSameDT=off
  Scope2 : Scope
  Scope7 : Scope  NumInputPorts=2
  WinDows Sector : Subsystem
  ZC_TimeOut_Juge : Subsystem
  n_est_compute : Subsystem
  Fault Memory1 : Outport
  Commutation Pulse : Outport  Port=2
  StepStart : Outport  Port=3
  t_sector : Outport  Port=4
  T60 : Outport  Port=5
  Open Loop Pulse1 : Outport  Port=6
  BlankingDone : Outport  Port=7
  ClosedMode Next : Outport  Port=8
  n_est_rpm1 : Outport  Port=9
  wires:
  Open Loop Pulse/1 -> Closed Loop Pulse/1(Open Loop Pulse)
  Step/1 -> Relational Operator/2, Previous Step/1
  ClosedMode Memory/1 -> ClosedModeStartSet/1(Open Loop Pulse), ZC_TimeOut_Juge/3(ClosedMode旧状态), Open Loop Pulse1/1, Closed Loop Pulse/6(换相选择Switch控制), Closed Loop Pulse/4(ClosedMode旧状态)
  Discrete-Time Integrator/1 -> t_sector/1, Compare To Constant6/1  "t_sector"
  Constant2/1 -> Discrete-Time Integrator/1
  ZC Accept/1 -> Closed Loop Pulse/5(ZC Accept)
  Closed Loop Pulse/1(T60) -> ZC_TimeOut_Juge/2(T60), Scope2/1, n_est_compute/1(In1), T60/1
  DetectEnable/1 -> WinDows Sector/3(DetectEnable), Closed Loop Pulse/2(Detect Enable)
  Tref/1 -> Closed Loop Pulse/7(Tref)
  Closed Loop Pulse/2(ClosedMode Next) -> ClosedMode Memory/1, ClosedMode Next/1
  Relational Operator/1 -> Discrete-Time Integrator/2, WinDows Sector/1(StepStart1), Closed Loop Pulse/8(StepStart), StepStart/1  "StepStart"
  Previous Step/1 -> Relational Operator/1
  Compare To Constant6/1 -> Closed Loop Pulse/3(Blanking Done), BlankingDone/1  "BlankingDone"
  Fault Memory/1 -> Fault Memory1/1, ClosedModeStartSet/3(Fault Memory), Closed Loop Pulse/9(Fault), Scope7/1
  ClosedModeStartSet/1(Fault Data) -> Fault Memory/1
  Closed Loop Pulse/3(Commutation Pulse) -> Commutation Pulse/1
  n_est_compute/1(n_est_rpm1) -> n_est_rpm1/1
  Closed Loop Pulse/4(Time Since ZC) -> ZC_TimeOut_Juge/1(Closed Loop Pulse)
  ZC_TimeOut_Juge/1(Is ZC TimeOut?) -> ClosedModeStartSet/2(ZC Timeout)
  WinDows Sector/1(WindowsOK) -> Scope7/2, Closed Loop Pulse/10(BadSector)
  ZC Seen Memory/1 -> WinDows Sector/2(In9)

== system six_stepItext/Subsystem/ZC Closed&Detect/Detect ==
  StepStart : Inport
  BlankingDone : Inport  Port=2
  DetectEnable : Inport  Port=3
  StepStart1 : Inport  Port=4
  ExpectedEdge : Inport  Port=5
  WindowsOK : Inport  Port=6
  ZC Positive SideData : Inport  Port=7
  Allow_detect : Subsystem
  Real_ZERO_Detect : Subsystem
  Armed : Outport
  ZCPulse : Outport  Port=2
  ZC Seen Memory : Outport  Port=3
  wires:
  ZC Positive SideData/1 -> Real_ZERO_Detect/2(ZC Negative SideData), Real_ZERO_Detect/1(ZC Positive SideData), Allow_detect/5(ZC Positive ArmData), Allow_detect/4(ZC Negative ArmData)
  ExpectedEdge/1 -> Real_ZERO_Detect/3(ExpectedEdge), Allow_detect/1(ExpectedEdge)
  DetectEnable/1 -> Real_ZERO_Detect/8(Detect Enable)
  BlankingDone/1 -> Real_ZERO_Detect/5(BlankingDone), Allow_detect/2(BlankingDone)
  StepStart/1 -> Real_ZERO_Detect/7(StepStart)
  Allow_detect/2(ZC Armed MemoryData) -> Real_ZERO_Detect/4(ZC Armed Memory)
  StepStart1/1 -> Allow_detect/3(StepStart)
  Allow_detect/1(Armed) -> Armed/1
  WindowsOK/1 -> Real_ZERO_Detect/6(WindowOK)
  Real_ZERO_Detect/2(ZC Seen Memory) -> ZC Seen Memory/1
  Real_ZERO_Detect/1(ZC Accept) -> ZCPulse/1  "ZCPulse"

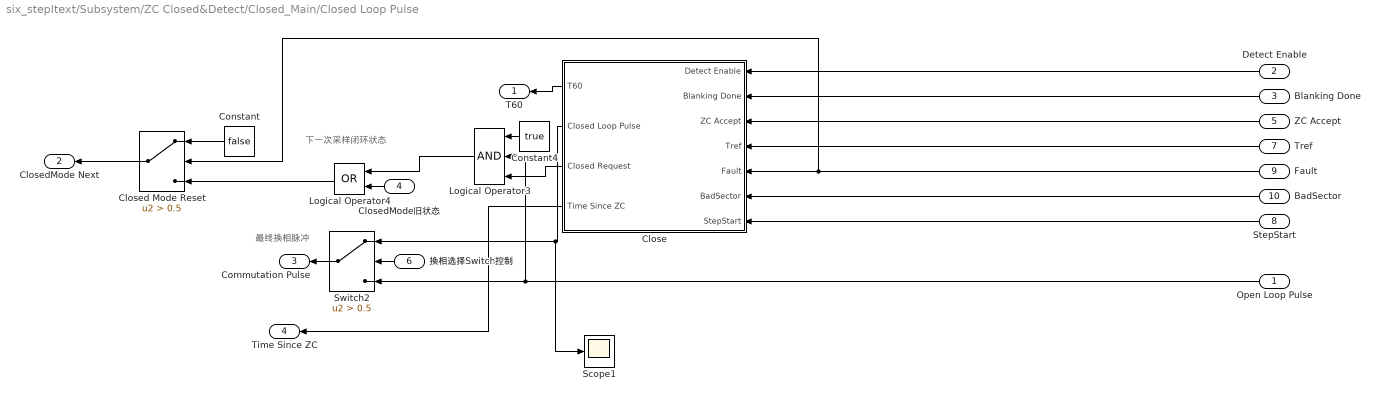
== system six_stepItext/Subsystem/ZC Closed&Detect/Closed_Main/Closed Loop Pulse ==
  note: 下一次采样闭环状态
  note: 最终换相脉冲
  Open Loop Pulse : Inport
  Detect Enable : Inport  Port=2
  Blanking Done : Inport  Port=3
  ClosedMode旧状态 : Inport  Port=4
  ZC Accept : Inport  Port=5
  换相选择Switch控制 : Inport  Port=6
  Tref : Inport  Port=7
  StepStart : Inport  Port=8
  Fault : Inport  Port=9
  BadSector : Inport  Port=10
  Close : Subsystem
  Closed Mode Reset : Switch  Criteria=u2 > Threshold  Threshold=0.5  SaturateOnIntegerOverflow=off  InputSameDT=off
  Constant : Constant  Value=false
  Constant4 : Constant  Value=true
  Logical Operator3 : Logic  Inputs=3  AllPortsSameDT=off  OutDataTypeStr=boolean
  Logical Operator4 : Logic  Operator=OR  AllPortsSameDT=off  OutDataTypeStr=boolean
  Scope1 : Scope
  Switch2 : Switch  Criteria=u2 > Threshold  Threshold=0.5  SaturateOnIntegerOverflow=off  InputSameDT=off
  T60 : Outport
  ClosedMode Next : Outport  Port=2
  Commutation Pulse : Outport  Port=3
  Time Since ZC : Outport  Port=4
  wires:
  Switch2/1 -> Commutation Pulse/1
  Open Loop Pulse/1 -> Logical Operator3/2, Switch2/3
  Detect Enable/1 -> Close/1(Detect Enable)
  ZC Accept/1 -> Close/3(ZC Accept)
  Close/2(Closed Loop Pulse) -> Scope1/1, Switch2/1
  Logical Operator3/1 -> Logical Operator4/1
  Blanking Done/1 -> Close/2(Blanking Done)
  Logical Operator4/1 -> Closed Mode Reset/3
  换相选择Switch控制/1 -> Switch2/2
  Close/1(T60) -> T60/1
  ClosedMode旧状态/1 -> Logical Operator4/2
  Tref/1 -> Close/4(Tref)
  Fault/1 -> Closed Mode Reset/2, Close/5(Fault)
  BadSector/1 -> Close/6(BadSector)
  Close/3(Closed Request) -> Logical Operator3/3
  StepStart/1 -> Close/7(StepStart)
  Constant4/1 -> Logical Operator3/1
  Close/4(Time Since ZC) -> Time Since ZC/1
  Constant/1 -> Closed Mode Reset/1
  Closed Mode Reset/1 -> ClosedMode Next/1

== system six_stepItext/Subsystem/ZC Closed&Detect/Closed_Main/ClosedModeStartSet ==
  Open Loop Pulse : Inport
  ZC Timeout : Inport  Port=2
  Fault Memory : Inport  Port=3
  Clock1 : Clock
  Fault Latch OR : Logic  Operator=OR  Inputs=3  AllPortsSameDT=off  OutDataTypeStr=boolean
  Not Closed Mode : Logic  Operator=NOT  AllPortsSameDT=off  OutDataTypeStr=boolean
  Startup Time Exceeded : simulink/Logic and Bit Operations/Compare To Constant  relop=>  const=7  OutDataTypeStr=boolean
  Startup Timeout : Logic  AllPortsSameDT=off  OutDataTypeStr=boolean
  Fault Data : Outport
  wires:
  Clock1/1 -> Startup Time Exceeded/1
  Startup Time Exceeded/1 -> Startup Timeout/1
  ZC Timeout/1 -> Fault Latch OR/2
  Startup Timeout/1 -> Fault Latch OR/1
  Not Closed Mode/1 -> Startup Timeout/2
  Open Loop Pulse/1 -> Not Closed Mode/1
  Fault Memory/1 -> Fault Latch OR/3
  Fault Latch OR/1 -> Fault Data/1

== system six_stepItext/Subsystem/ZC Closed&Detect/Closed_Main/WinDows Sector ==
  StepStart1 : Inport
  In9 : Inport  Port=2
  DetectEnable : Inport  Port=3
  Bad Sector : Logic  Inputs=3  AllPortsSameDT=off  OutDataTypeStr=boolean
  Not ZC in Sector : Logic  Operator=NOT  AllPortsSameDT=off  OutDataTypeStr=boolean
  WindowsOK : Outport
  wires:
  DetectEnable/1 -> Bad Sector/3
  In9/1 -> Not ZC in Sector/1
  Not ZC in Sector/1 -> Bad Sector/2  "WindowsOK"
  Bad Sector/1 -> WindowsOK/1  "WindowsOK"
  StepStart1/1 -> Bad Sector/1

== system six_stepItext/Subsystem/ZC Closed&Detect/Closed_Main/ZC_TimeOut_Juge ==
  Closed Loop Pulse : Inport
  T60 : Inport  Port=2
  ClosedMode旧状态 : Inport  Port=3
  ZC Timeout : Logic  AllPortsSameDT=off  OutDataTypeStr=boolean
  ZC Timeout Compare : RelationalOperator  Operator=>  OutDataTypeStr=boolean  RndMeth=Simplest  InputSameDT=off
  ZC Timeout Limit : Gain  Gain=2
  Is ZC TimeOut? : Outport
  wires:
  T60/1 -> ZC Timeout Limit/1
  ZC Timeout/1 -> Is ZC TimeOut?/1
  ZC Timeout Compare/1 -> ZC Timeout/1
  ZC Timeout Limit/1 -> ZC Timeout Compare/2
  ClosedMode旧状态/1 -> ZC Timeout/2
  Closed Loop Pulse/1 -> ZC Timeout Compare/1

== system six_stepItext/Subsystem/ZC Closed&Detect/Closed_Main/n_est_compute ==
  In1 : Inport
  Constant1 : Constant  Value=1.6667
  Scope : Scope
  n_est_rpm : Product  Inputs=*/
  n_est_rpm1 : Outport
  wires:
  n_est_rpm/1 -> n_est_rpm1/1, Scope/1  "n_est_rpm"
  In1/1 -> n_est_rpm/2
  Constant1/1 -> n_est_rpm/1
